simulink model "ballPlane"  (R2026a)
settings: Solver=ode45  StopTime=6.0  MaxStep=0.005
InitFcn:
  | ballPlane_param
values from neighbouring files (symbols this model uses):
  b = 0.005    [ballPlane_param.m]
  dx_init = 0.0    (= 0)    [ballPlane_param.m]
  g = 9.81    [ballPlane_param.m]
  m = 0.05    [ballPlane_param.m]
  tau_m = 0.05    [ballPlane_param.m]
  theta_init = 0.0    (= 0)    [ballPlane_param.m]
  theta_max = 20 * pi / 180    (= 0.349065850399)    [ballPlane_param.m]
  x_init = 0.0    (= 0)    [ballPlane_param.m]
  x_max = L / 2    (= 0.3)    [ballPlane_param.m]
  x_min = -L / 2    (= -0.3)    [ballPlane_param.m]
undefined symbols (not defined in the file or in its folder): Kd, Ki, Kp
settings Model: Creator=juraj  LastModifiedBy=juraj

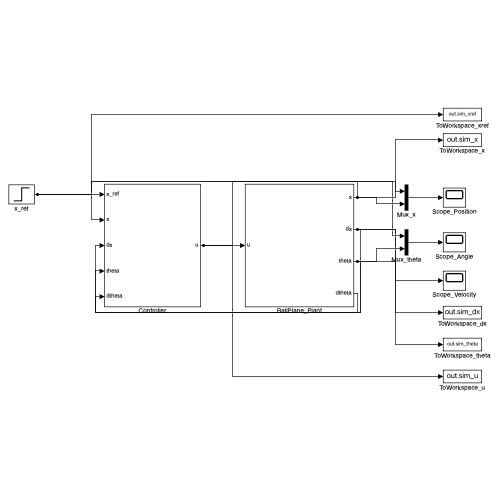
[thumbnail: Simulink's stored preview of the top-level diagram]
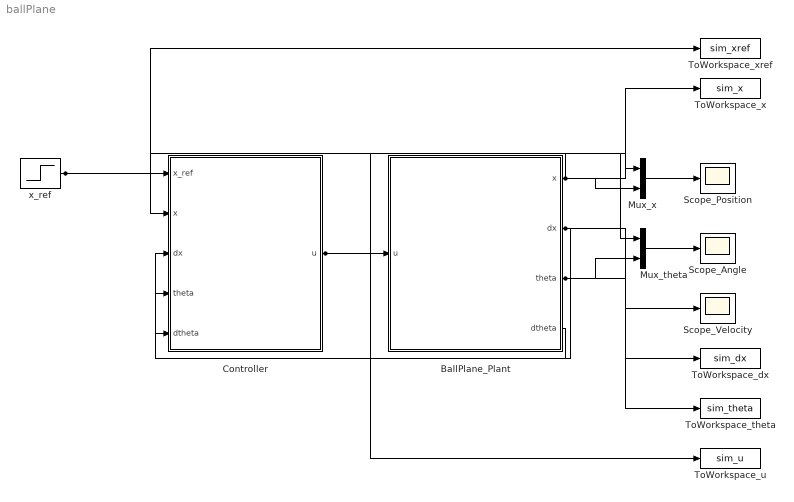
== system ballPlane ==
  BallPlane_Plant : Subsystem
  Controller : Subsystem
  Mux_theta : Mux  Inputs=2
  Mux_x : Mux  Inputs=2
  Scope_Angle : Scope
  Scope_Position : Scope
  Scope_Velocity : Scope
  ToWorkspace_dx : ToWorkspace  VariableName=sim_dx  SaveFormat=Timeseries  SampleTime=-1
  ToWorkspace_theta : ToWorkspace  VariableName=sim_theta  SaveFormat=Timeseries  SampleTime=-1
  ToWorkspace_u : ToWorkspace  VariableName=sim_u  SaveFormat=Timeseries  SampleTime=-1
  ToWorkspace_x : ToWorkspace  VariableName=sim_x  SaveFormat=Timeseries  SampleTime=-1
  ToWorkspace_xref : ToWorkspace  VariableName=sim_xref  SaveFormat=Timeseries  SampleTime=-1
  x_ref : Step  Time=1.0  InitialValue=0.0  FinalValue=0.15  SampleTime=0
  wires:
  x_ref/1 -> Controller/1(x_ref), Mux_x/1, ToWorkspace_xref/1
  Controller/1(u) -> BallPlane_Plant/1(u), Mux_theta/1, ToWorkspace_u/1
  BallPlane_Plant/1(x) -> Controller/2(x), Mux_x/2, ToWorkspace_x/1
  BallPlane_Plant/2(dx) -> Controller/3(dx), Scope_Velocity/1, ToWorkspace_dx/1
  BallPlane_Plant/3(theta) -> Controller/4(theta), Mux_theta/2, ToWorkspace_theta/1
  BallPlane_Plant/4(dtheta) -> Controller/5(dtheta)
  Mux_x/1 -> Scope_Position/1
  Mux_theta/1 -> Scope_Angle/1

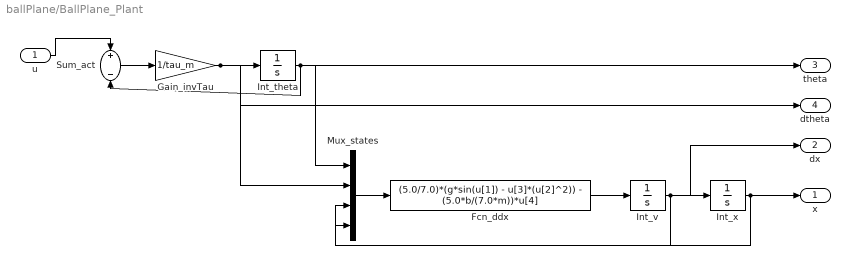
== system ballPlane/BallPlane_Plant ==
  u : Inport
  Fcn_ddx : Fcn  Expr=(5.0/7.0)*(g*sin(u[1]) - u[3]*(u[2]^2)) - (5.0*b/(7.0*m))*u[4]
  Gain_invTau : Gain  Gain=1/tau_m
  Int_theta : Integrator  InitialCondition=theta_init  LimitOutput=on  UpperSaturationLimit=theta_max  LowerSaturationLimit=-theta_max
  Int_v : Integrator  InitialCondition=dx_init
  Int_x : Integrator  InitialCondition=x_init  LimitOutput=on  UpperSaturationLimit=x_max  LowerSaturationLimit=x_min
  Mux_states : Mux
  Sum_act : Sum  Inputs=+-
  x : Outport
  dx : Outport  Port=2
  theta : Outport  Port=3
  dtheta : Outport  Port=4
  wires:
  u/1 -> Sum_act/1
  Sum_act/1 -> Gain_invTau/1
  Gain_invTau/1 -> Int_theta/1, Mux_states/2, dtheta/1
  Int_theta/1 -> Sum_act/2, Mux_states/1, theta/1
  Int_x/1 -> Mux_states/3, x/1
  Int_v/1 -> Mux_states/4, Int_x/1, dx/1
  Mux_states/1 -> Fcn_ddx/1
  Fcn_ddx/1 -> Int_v/1

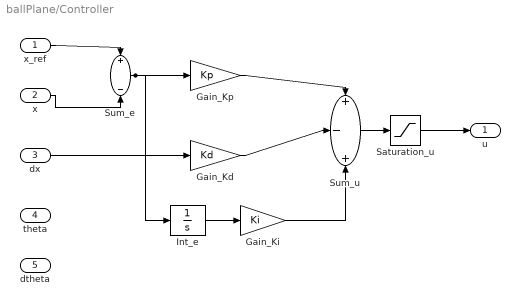
== system ballPlane/Controller ==
  x_ref : Inport
  x : Inport  Port=2
  dx : Inport  Port=3
  theta : Inport  Port=4
  dtheta : Inport  Port=5
  Gain_Kd : Gain  Gain=Kd
  Gain_Ki : Gain  Gain=Ki
  Gain_Kp : Gain  Gain=Kp
  Int_e : Integrator  LimitOutput=on  UpperSaturationLimit=0.5  LowerSaturationLimit=-0.5
  Saturation_u : Saturate  UpperLimit=theta_max  LowerLimit=-theta_max
  Sum_e : Sum  Inputs=+-
  Sum_u : Sum  Inputs=+-+
  u : Outport
  wires:
  x_ref/1 -> Sum_e/1
  x/1 -> Sum_e/2
  Sum_e/1 -> Gain_Kp/1, Int_e/1
  dx/1 -> Gain_Kd/1
  Int_e/1 -> Gain_Ki/1
  Gain_Kp/1 -> Sum_u/1
  Gain_Kd/1 -> Sum_u/2
  Gain_Ki/1 -> Sum_u/3
  Sum_u/1 -> Saturation_u/1
  Saturation_u/1 -> u/1
